simulink model "si_fuzzy_pid_tank"  (R2025b)
settings: Solver=FixedStepDiscrete  StartTime=0.0  StopTime=80  FixedStep=.2  RelTol=1e-3
model workspace (MAT data in the model file):
  dt = 0.2
  model.kind = 'rbf'
  model.centers = [0.374540118847  0.69816171402; 0.95071430641  0.536096366344; 0.731993941811  0.309527616286; 0.598658484197  0.813795019707; 0.156018640442  0.684731172554; 0.155994520336  0.162616939345; 0.0580836121682  0.910927184494; 0.866176145775  0.822537242923; 0.601115011743  0.949799913292; 0.708072577796  0.725719508388; 0.0205844942958  0.613415195936; 0.969909852162  0.418243036291; 0.8324426408  0.932728483354; 0.212339110678  0.8660638895; 0.181824967207  0.0452186701062; 0.183404509853  0.0263669744973; 0.30424224296  0.376463366878; 0.524756431632  0.810553330782; 0.431945018642  0.987276129315; 0.291229140198  0.150416891104; 0.611852894722  0.594130715352; 0.139493860652  0.380890856631; 0.292144648535  0.969914397815; 0.366361843294  0.842118923136; 0.456069984217  0.838328704711]
  model.width = 0.3
  model.weights = [0.947882905436; -4.30991473624; -0.345821249434; -0.23987212642; -5.0913471804; -4.45040594909; -29.9120883058; -2.95166063721; 1.69110200234; -4.93369717649; -3.97957792292; -2.12801913243; 0.55445060854; 0.200554032619; 16.8853229202; 142.870250847; -118.128771749; 0.43077208105; 28.7009383642; 10.9471358908; -2.96117817166; 0.997908698828; 9.44779249754; -13.2754293471; 2.81376842779; -25.6534276996]
  p.dt = 0.2
  p.filter_time = 0.5
  reference_data = [0 0.2 0.4 0.6 0.8 1 1.2 1.4 1.6 1.8 2 2.2 ... (802 elements, 401x2)]
settings Model: Creator=runner  LastModifiedBy=runner

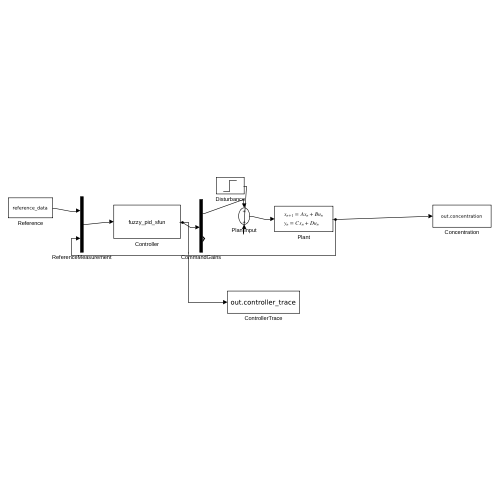
[thumbnail: Simulink's stored preview of the top-level diagram]
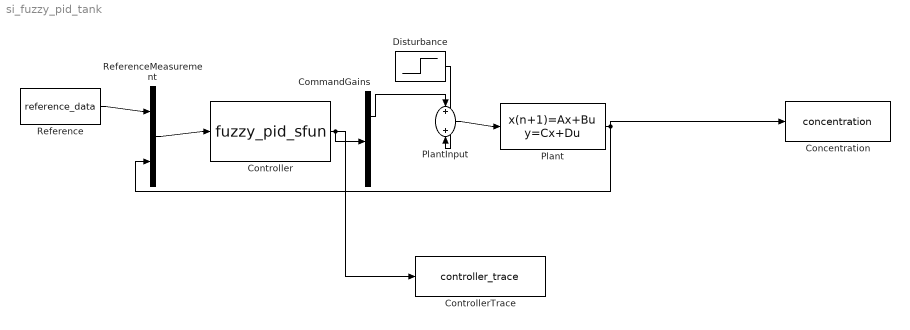
== system si_fuzzy_pid_tank ==
  CommandGains : Demux  Outputs=[1 4]
  Concentration : ToWorkspace  VariableName=concentration  SaveFormat=Structure With Time  SampleTime=-1
  Controller : S-Function  FunctionName=fuzzy_pid_sfun  Parameters=p  SFunctionDeploymentMode=off  EnableBusSupport=off
  ControllerTrace : ToWorkspace  VariableName=controller_trace  SaveFormat=Structure With Time  SampleTime=-1
  Disturbance : Step  Time=45  After=.08  SampleTime=dt
  Plant : DiscreteStateSpace  A=exp(-dt/10)  B=1-exp(-dt/10)  D=0  InitialCondition=.35  SampleTime=dt
  PlantInput : Sum
  Reference : FromWorkspace  VariableName=reference_data  SampleTime=dt  Interpolate=off  OutputAfterFinalValue=Holding final value
  ReferenceMeasurement : Mux  Inputs=2
  wires:
  Controller/1 -> CommandGains/1, ControllerTrace/1
  CommandGains/1 -> PlantInput/1
  Disturbance/1 -> PlantInput/2
  PlantInput/1 -> Plant/1
  Reference/1 -> ReferenceMeasurement/1
  Plant/1 -> ReferenceMeasurement/2, Concentration/1
  ReferenceMeasurement/1 -> Controller/1
